simulink model "hrg_tdm_shared"  (R2025a)
settings: Solver=FixedStepDiscrete  StartTime=0.0  StopTime=c.duration  FixedStep=c.Ts  RelTol=1e-3
model workspace (MAT data in the model file):
  c.reuse = 1
  c.Ts = 6.25e-06
  c.w = 6283.18530718
  c.omega = 0.5
  c.duration = 1.2
  c.B = 0.276990961962
  c.driveEnd = 160
  c.senseStart = 192
  c.validStart = 272
  c.validEnd = 432
  c.frame = 480
  c.n = 160
  c.adcStep = 1.90734863281e-06
  c.adcMax = 0.999998092651
  c.adcMin = -1
  c.dacStep = 7.62939453125e-06
  c.dacMax = 0.999992370605
  c.dacMin = -1
  c.minEnergy = 0.0004
  c.minLinearity = 0.1
  c.agc = 12.5663706144
  c.gamma = 0.314159265359
  c.quad = 25.1327412287
  c.forceScale = 0.342719198573
  c.startCommand = [0; 0; 0; 0]
  c.pickoff = [0  0  0  0  0  0  0  0  0  0  0.1  0; 0  0  0  0  0  0  0  0  0  0  0  0.1]
  c.electrode = [0  0  0  0  0  0  6.28318530718e-05  0  0  0  0  0; 0  0  0  0  0  0  0  6.28318530718e-05  0  0  0  0]
  c.motion = [1  0  0  0  0  0  0  0  0  0  0  0; 0  1  0  0  0  0  0  0  0  0  0  0]
  c.Ad = [0.99922903725  -8.89767021045e-10  0.0392597386726  6.79661603948e-08  1.94082542713e-06  -5.91938484731e-08  0  0  0  0  0  0; 8.89767021045e-10  0.99922903725  -6.79661603948e-08  0.0392597386726  3.88142106306e-08  2.13106904302e-06  0  0  0  0  0  0; -0.0392597386726  -6.79661603967e-08  0.99922511127  3.46059382687e-06  9.39460935417e-05  -2.88897470742e-06  0  0  0  0  0  0; 6.79661603967e-08  -0.0392597386726  -3.46059382687e-06  0.99922511127  1.87875070496e-06  0.000104009857967  0  0  0  0  0  0; 0  0  0  0  0.731615628947  0  0  0  0  0  0  0; 0  0  0  0  0  0.770730381232  0  0  0  0  0  0; 0  0  0  0  11644.024379  0  0  0  0  0  0  0; 0  0  0  0  0  12266.5549964  0  0  0  0  0  0; 0  0  0  0  0  0  0  0  0.999937501953  0  0  0; 0  0  0  0  0  0  0  0  0  0.999937501953  0  0; 0  0  0  0  0  0  0  0  0.544042667727  0.0136010666932  0.455938127766  0; 0  0  0  0  0  0  0  0  -0.00760186665633  0.527062754839  0  0.493191201703]
  c.Bd = [2.07333228059e-07  -5.2482321733e-09; 4.14648229472e-09  1.8894232541e-07; 1.54445980203e-05  -3.92541399381e-07; 3.08873674204e-07  1.41320905111e-05; 0.268384371053  0; 0  0.229269618768; 4271.46993018  0; 0  3648.93931278; 0  0; 0  0; 0  0; 0  0]
  c.Af = [0.999229037252  -8.89767017797e-10  0.0392597384416  6.79661599867e-08  0  0  1.0729670464e-10  1.28007724625e-16  0  0  0  0; 8.89767017797e-10  0.999229037252  -6.79661599867e-08  0.0392597384416  0  0  -1.28007724618e-16  1.07296704251e-10  0  0  0  0; -0.0392597384416  -6.79661599886e-08  0.999225094196  3.46059378613e-06  0  0  5.10992633221e-09  9.4589441098e-15  0  0  0  0; 6.79661599886e-08  -0.0392597384416  -3.46059378613e-06  0.999225094196  0  0  -9.45894412526e-15  5.10992631239e-09  0  0  0  0; 0  0  0  0  0.731615628947  0  0  0  0  0  0  0; 0  0  0  0  0  0.770730381232  0  0  0  0  0  0; 0.107296704687  1.28007724925e-07  -5.10992633457  -9.45894414256e-06  0  0  0.65924020331  -1.83788136052e-14  0  0  0  0; -1.28007724925e-07  0.107296704687  9.45894414256e-06  -5.10992633457  0  0  1.83788135899e-14  0.65924020331  0  0  0  0; 0  0  0  0  0  0  0  0  0.731615628947  0  0  0; 0  0  0  0  0  0  0  0  0  0.731615628947  0  0; 0  0  0  0  0  0  0  0  0.457850378529  0.0114462594632  0.455938127766  0; 0  0  0  0  0  0  0  0  -0.00641037388191  0.444452589146  0  0.493191201703]
  c.As = [0.999229037251  -8.89767019419e-10  0.0392597385829  6.7966160211e-08  0  0  3.299223447e-11  4.96927081282e-17  0  0  0  0; 8.89767019419e-10  0.999229037251  -6.7966160211e-08  0.0392597385829  0  0  -4.9692697e-17  3.29922429769e-11  0  0  0  0; -0.0392597385829  -6.79661602128e-08  0.99922510602  3.46059381106e-06  0  0  9.97502201431e-10  2.90830921925e-15  0  0  0  0; 6.79661602128e-08  -0.0392597385829  -3.46059381106e-06  0.99922510602  0  0  -2.90830846447e-15  9.97502498523e-10  0  0  0  0; 0  0  0  0  0.731615628947  0  0  0  0  0  0  0; 0  0  0  0  0  0.770730381232  0  0  0  0  0  0; 0.0329922423735  4.96927093775e-08  -0.997502477449  -2.90830923686e-06  0  0  0.00193045194409  -2.36252148067e-15  0  0  0  0; -4.96927093775e-08  0.0329922423735  2.90830923686e-06  -0.997502477449  0  0  2.36252088829e-15  0.00193045194409  0  0  0  0; 0.000563655894429  5.77530332379e-10  -0.0329913452873  -4.96917902079e-08  0  0  0.00627072528027  -3.48479736566e-17  0.999937501953  0  0  0; -5.77530332379e-10  0.000563655894429  4.96917902079e-08  -0.0329913452873  0  0  3.4847965996e-17  0.00627072528027  0  0.999937501953  0  0; 0.000110797632844  2.77002999452e-06  -0.00905716494292  -0.000226438897931  0  0  0.00300835962776  7.52089906939e-05  0.544042667727  0.0136010666932  0.455938127766  0; -1.51991580376e-06  0.000105374968441  0.000124839418396  -0.00865488875584  0  0  -4.18601716323e-05  0.00290230523317  -0.00760186665633  0.527062754839  0  0.493191201703]
  c.x0 = [0.276318298201; 0.116825502693; 0; 0; 0; 0; 0; 0; 0; 0; 0; 0]
  c.detect = [-9.99415152174  0.240237763684  -0.546724271016  0.0144774125637; -0.144146416179  -9.60951054736  -0.00788544621657  -0.579096502547; 0.546724271016  -0.0144774125637  -9.99415152174  0.240237763684; 0.00788544621657  0.579096502547  -0.144146416179  -9.60951054736]
  c.drive = [0.996850279412  0.0276902855392  0.14520184302  0.00403338452835; -0.018451056911  0.922552845551  -0.00315402594922  0.157701297461; -0.14520184302  -0.00403338452835  0.996850279412  0.0276902855392; 0.00315402594922  -0.157701297461  -0.018451056911  0.922552845551]
settings Model: Creator=Administrator  LastModifiedBy=Administrator

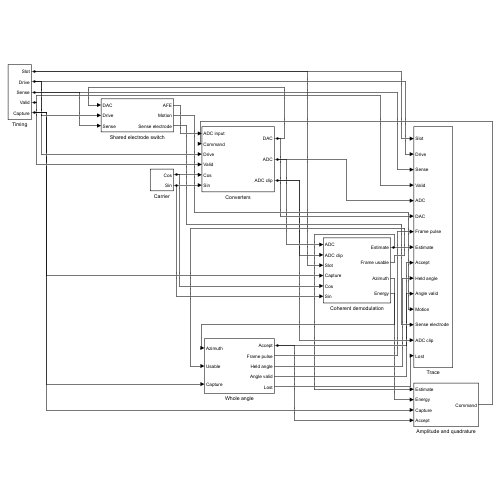
[thumbnail: Simulink's stored preview of the top-level diagram]
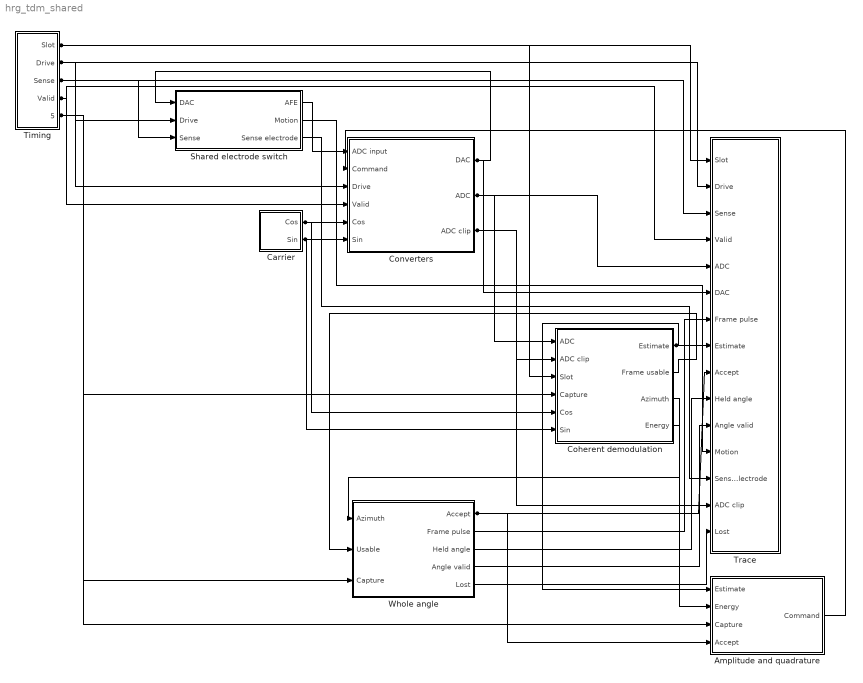
== system hrg_tdm_shared ==
  Amplitude and quadrature : Subsystem
  Carrier : Subsystem
  Coherent demodulation : Subsystem
  Converters : Subsystem
  Shared electrode switch : Subsystem
  Timing : Subsystem
  Trace : Subsystem
  Whole angle : Subsystem
  wires:
  Timing/1(Slot) -> Trace/1(Slot), Coherent demodulation/3(Slot)
  Timing/2(Drive) -> Trace/2(Drive), Converters/3(Drive), Shared electrode switch/2(Drive)
  Timing/3(Sense) -> Trace/3(Sense), Shared electrode switch/3(Sense)
  Coherent demodulation/2(Frame usable) -> Whole angle/2(Usable)
  Shared electrode switch/2(Motion) -> Trace/12(Motion)
  Shared electrode switch/1(AFE) -> Converters/1(ADC input)
  Carrier/2(Sin) -> Coherent demodulation/6(Sin), Converters/6(Sin)
  Timing/4(Valid) -> Converters/4(Valid), Trace/4(Valid)
  Whole angle/1(Accept) -> Trace/9(Accept), Amplitude and quadrature/4(Accept)
  Timing/5(Capture) -> Coherent demodulation/4(Capture), Amplitude and quadrature/3(Capture), Whole angle/3(Capture)
  Shared electrode switch/3(Sense electrode) -> Trace/13(Sense electrode)
  Carrier/1(Cos) -> Coherent demodulation/5(Cos), Converters/5(Cos)
  Converters/1(DAC) -> Shared electrode switch/1(DAC), Trace/6(DAC)
  Converters/2(ADC) -> Trace/5(ADC), Coherent demodulation/1(ADC)
  Converters/3(ADC clip) -> Trace/14(ADC clip), Coherent demodulation/2(ADC clip)
  Whole angle/2(Frame pulse) -> Trace/7(Frame pulse)
  Whole angle/3(Held angle) -> Trace/10(Held angle)
  Coherent demodulation/1(Estimate) -> Amplitude and quadrature/1(Estimate), Trace/8(Estimate)
  Whole angle/4(Angle valid) -> Trace/11(Angle valid)
  Whole angle/5(Lost) -> Trace/15(Lost)
  Coherent demodulation/3(Azimuth) -> Whole angle/1(Azimuth)
  Coherent demodulation/4(Energy) -> Amplitude and quadrature/2(Energy)
  Amplitude and quadrature/1(Command) -> Converters/2(Command)

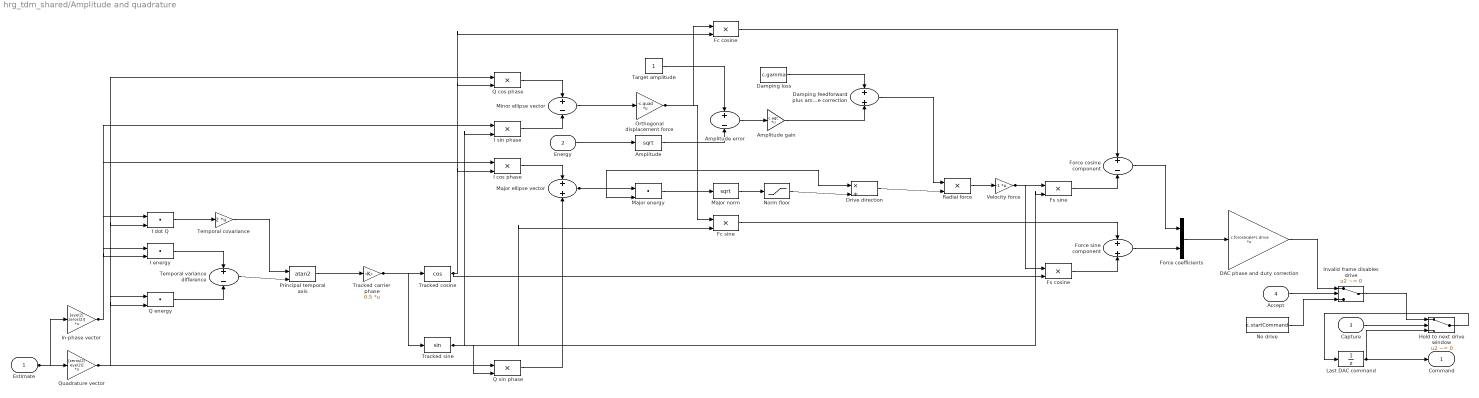
== system hrg_tdm_shared/Amplitude and quadrature ==
  Estimate : Inport
  Energy : Inport  Port=2
  Capture : Inport  Port=3
  Accept : Inport  Port=4
  Amplitude : Sqrt
  Amplitude error : Sum  Inputs=+-
  Amplitude gain : Gain  Gain=c.agc  Multiplication=Matrix(K*u)
  DAC phase and duty correction : Gain  Gain=c.forceScale*c.drive  Multiplication=Matrix(K*u)
  Damping feedforward plus amplitude correction : Sum
  Damping loss : Constant  Value=c.gamma
  Drive direction : Product  Inputs=*/
  Fc cosine : Product
  Fc sine : Product
  Force coefficients : Mux  Inputs=2
  Force cosine component : Sum  Inputs=+-
  Force sine component : Sum
  Fs cosine : Product
  Fs sine : Product
  Hold to next drive window : Switch  Criteria=u2 ~= 0  SaturateOnIntegerOverflow=off  InputSameDT=off
  I cos phase : Product
  I dot Q : DotProduct  OutDataTypeStr=Inherit: Inherit via internal rule
  I energy : DotProduct  OutDataTypeStr=Inherit: Inherit via internal rule
  I sin phase : Product
  In-phase vector : Gain  Gain=[eye(2) zeros(2)]  Multiplication=Matrix(K*u)
  Invalid frame disables drive : Switch  Criteria=u2 ~= 0  SaturateOnIntegerOverflow=off  InputSameDT=off
  Last DAC command : UnitDelay  InitialCondition=c.startCommand  SampleTime=c.Ts  HasFrameUpgradeWarning=on
  Major ellipse vector : Sum
  Major energy : DotProduct  OutDataTypeStr=Inherit: Inherit via internal rule
  Major norm : Sqrt
  Minor ellipse vector : Sum  Inputs=+-
  No drive : Constant  Value=c.startCommand
  Norm floor : Saturate  UpperLimit=inf  LowerLimit=1e-9
  Orthogonal displacement force : Gain  Gain=-c.quad  Multiplication=Matrix(K*u)
  Principal temporal axis : Trigonometry  Operator=atan2
  Q cos phase : Product
  Q energy : DotProduct  OutDataTypeStr=Inherit: Inherit via internal rule
  Q sin phase : Product
  Quadrature vector : Gain  Gain=[zeros(2) eye(2)]  Multiplication=Matrix(K*u)
  Radial force : Product
  Target amplitude : Constant
  Temporal covariance : Gain  Gain=2  Multiplication=Matrix(K*u)
  Temporal variance difference : Sum  Inputs=+-
  Tracked carrier phase : Gain  Gain=0.5  Multiplication=Matrix(K*u)
  Tracked cosine : Trigonometry  Operator=cos
  Tracked sine : Trigonometry
  Velocity force : Gain  Gain=-1  Multiplication=Matrix(K*u)
  Command : Outport
  wires:
  Estimate/1 -> In-phase vector/1, Quadrature vector/1
  Temporal covariance/1 -> Principal temporal axis/1
  I dot Q/1 -> Temporal covariance/1
  In-phase vector/1 -> I sin phase/1, I energy/1, I energy/2, I dot Q/1, I cos phase/1
  Amplitude gain/1 -> Damping feedforward plus amplitude correction/2
  Tracked carrier phase/1 -> Tracked cosine/1, Tracked sine/1
  Temporal variance difference/1 -> Principal temporal axis/2
  Minor ellipse vector/1 -> Orthogonal displacement force/1
  Quadrature vector/1 -> Q sin phase/1, Q cos phase/1, Q energy/1, Q energy/2, I dot Q/2
  Force coefficients/1 -> DAC phase and duty correction/1
  I energy/1 -> Temporal variance difference/1
  Q energy/1 -> Temporal variance difference/2
  Principal temporal axis/1 -> Tracked carrier phase/1
  Force sine component/1 -> Force coefficients/2
  Tracked cosine/1 -> Fc cosine/2, Fs cosine/2, Q cos phase/2, I cos phase/2
  Energy/1 -> Amplitude/1
  Tracked sine/1 -> Fc sine/2, Fs sine/2, I sin phase/2, Q sin phase/2
  No drive/1 -> Invalid frame disables drive/3
  Fs cosine/1 -> Force sine component/2
  Q cos phase/1 -> Minor ellipse vector/1
  Amplitude error/1 -> Amplitude gain/1
  I sin phase/1 -> Minor ellipse vector/2
  I cos phase/1 -> Major ellipse vector/1
  Q sin phase/1 -> Major ellipse vector/2
  DAC phase and duty correction/1 -> Invalid frame disables drive/1
  Major ellipse vector/1 -> Drive direction/1, Major energy/1, Major energy/2
  Capture/1 -> Hold to next drive window/2
  Fc cosine/1 -> Force cosine component/1
  Target amplitude/1 -> Amplitude error/1
  Orthogonal displacement force/1 -> Fc sine/1, Fc cosine/1
  Amplitude/1 -> Amplitude error/2
  Major energy/1 -> Major norm/1
  Major norm/1 -> Norm floor/1
  Fc sine/1 -> Force sine component/1
  Force cosine component/1 -> Force coefficients/1
  Damping loss/1 -> Damping feedforward plus amplitude correction/1
  Norm floor/1 -> Drive direction/2
  Damping feedforward plus amplitude correction/1 -> Radial force/1
  Drive direction/1 -> Radial force/2
  Radial force/1 -> Velocity force/1
  Velocity force/1 -> Fs sine/1, Fs cosine/1
  Fs sine/1 -> Force cosine component/2
  Accept/1 -> Invalid frame disables drive/2
  Invalid frame disables drive/1 -> Hold to next drive window/1
  Last DAC command/1 -> Hold to next drive window/3, Command/1
  Hold to next drive window/1 -> Last DAC command/1

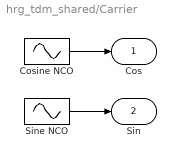
== system hrg_tdm_shared/Carrier ==
  Cosine NCO : Sin  Frequency=c.w  Phase=pi/2  SampleTime=c.Ts
  Sine NCO : Sin  Frequency=c.w  SampleTime=c.Ts
  Cos : Outport
  Sin : Outport  Port=2
  wires:
  Cosine NCO/1 -> Cos/1
  Sine NCO/1 -> Sin/1

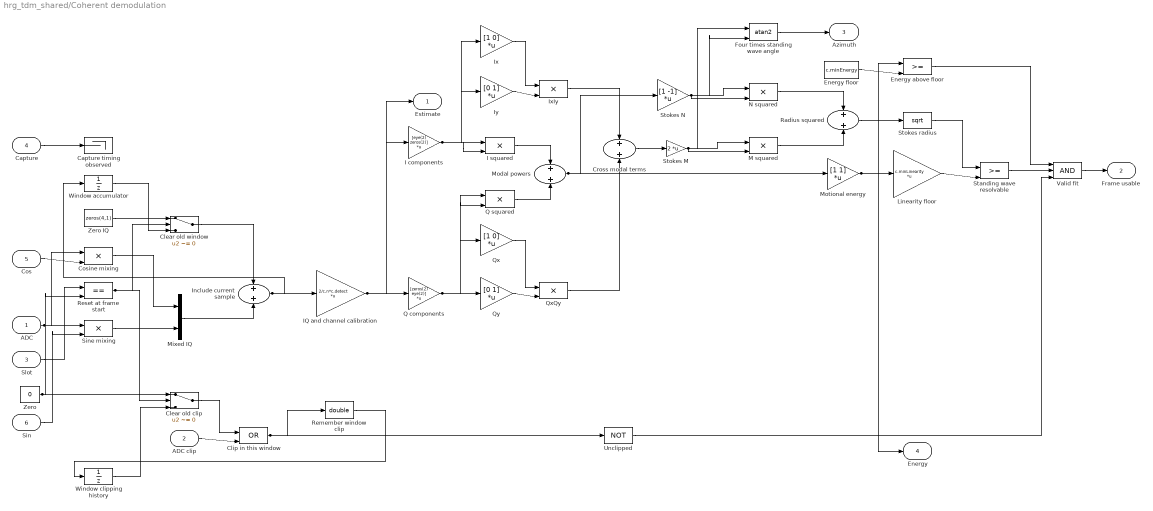
== system hrg_tdm_shared/Coherent demodulation ==
  ADC : Inport
  ADC clip : Inport  Port=2
  Slot : Inport  Port=3
  Capture : Inport  Port=4
  Cos : Inport  Port=5
  Sin : Inport  Port=6
  Capture timing observed : Terminator
  Clear old clip : Switch  Criteria=u2 ~= 0  SaturateOnIntegerOverflow=off  InputSameDT=off
  Clear old window : Switch  Criteria=u2 ~= 0  SaturateOnIntegerOverflow=off  InputSameDT=off
  Clip in this window : Logic  Operator=OR  AllPortsSameDT=off  OutDataTypeStr=boolean
  Cosine mixing : Product
  Cross modal terms : Sum
  Energy above floor : RelationalOperator  OutDataTypeStr=boolean  RndMeth=Simplest  InputSameDT=off
  Energy floor : Constant  Value=c.minEnergy
  Four times standing wave angle : Trigonometry  Operator=atan2
  I components : Gain  Gain=[eye(2) zeros(2)]  Multiplication=Matrix(K*u)
  I squared : Product
  IQ and channel calibration : Gain  Gain=2/c.n*c.detect  Multiplication=Matrix(K*u)
  Include current sample : Sum
  Ix : Gain  Gain=[1 0]  Multiplication=Matrix(K*u)
  IxIy : Product
  Iy : Gain  Gain=[0 1]  Multiplication=Matrix(K*u)
  Linearity floor : Gain  Gain=c.minLinearity  Multiplication=Matrix(K*u)
  M squared : Product
  Mixed IQ : Mux  Inputs=2
  Modal powers : Sum
  Motional energy : Gain  Gain=[1 1]  Multiplication=Matrix(K*u)
  N squared : Product
  Q components : Gain  Gain=[zeros(2) eye(2)]  Multiplication=Matrix(K*u)
  Q squared : Product
  Qx : Gain  Gain=[1 0]  Multiplication=Matrix(K*u)
  QxQy : Product
  Qy : Gain  Gain=[0 1]  Multiplication=Matrix(K*u)
  Radius squared : Sum
  Remember window clip : DataTypeConversion  OutDataTypeStr=double  SaturateOnIntegerOverflow=off  RndMeth=Floor
  Reset at frame start : RelationalOperator  Operator===  OutDataTypeStr=boolean  RndMeth=Simplest  InputSameDT=off
  Sine mixing : Product
  Standing wave resolvable : RelationalOperator  OutDataTypeStr=boolean  RndMeth=Simplest  InputSameDT=off
  Stokes M : Gain  Gain=2  Multiplication=Matrix(K*u)
  Stokes N : Gain  Gain=[1 -1]  Multiplication=Matrix(K*u)
  Stokes radius : Sqrt
  Unclipped : Logic  Operator=NOT  Inputs=1  AllPortsSameDT=off  OutDataTypeStr=boolean
  Valid fit : Logic  Inputs=3  AllPortsSameDT=off  OutDataTypeStr=boolean
  Window accumulator : UnitDelay  InitialCondition=zeros(4,1)  SampleTime=c.Ts  HasFrameUpgradeWarning=on
  Window clipping history : UnitDelay  SampleTime=c.Ts  HasFrameUpgradeWarning=on
  Zero : Constant  Value=0
  Zero IQ : Constant  Value=zeros(4,1)
  Estimate : Outport
  Frame usable : Outport  Port=2
  Azimuth : Outport  Port=3
  Energy : Outport  Port=4
  wires:
  Slot/1 -> Reset at frame start/1
  I components/1 -> I squared/2, Ix/1, Iy/1, I squared/1
  Clear old clip/1 -> Clip in this window/1
  Capture/1 -> Capture timing observed/1
  I squared/1 -> Modal powers/1
  Cos/1 -> Cosine mixing/2
  Zero/1 -> Clear old clip/1, Reset at frame start/2
  Stokes radius/1 -> Standing wave resolvable/1
  ADC/1 -> Cosine mixing/1, Sine mixing/1
  ADC clip/1 -> Clip in this window/2
  Sin/1 -> Sine mixing/2
  Window accumulator/1 -> Clear old window/3
  Cross modal terms/1 -> Stokes M/1
  Zero IQ/1 -> Clear old window/1
  Cosine mixing/1 -> Mixed IQ/1
  Reset at frame start/1 -> Clear old clip/2, Clear old window/2
  Standing wave resolvable/1 -> Valid fit/2
  Sine mixing/1 -> Mixed IQ/2
  Window clipping history/1 -> Clear old clip/3
  Clear old window/1 -> Include current sample/1
  Mixed IQ/1 -> Include current sample/2
  Motional energy/1 -> Energy above floor/1, Linearity floor/1, Energy/1
  Include current sample/1 -> Window accumulator/1, IQ and channel calibration/1
  Clip in this window/1 -> Unclipped/1, Remember window clip/1
  IQ and channel calibration/1 -> I components/1, Q components/1, Estimate/1
  Remember window clip/1 -> Window clipping history/1
  Q components/1 -> Q squared/1, Qy/1, Qx/1, Q squared/2
  Unclipped/1 -> Valid fit/3
  Ix/1 -> IxIy/1
  Iy/1 -> IxIy/2
  Q squared/1 -> Modal powers/2
  Qx/1 -> QxQy/1
  Linearity floor/1 -> Standing wave resolvable/2
  M squared/1 -> Radius squared/2
  Qy/1 -> QxQy/2
  IxIy/1 -> Cross modal terms/1
  Modal powers/1 -> Motional energy/1, Stokes N/1
  QxQy/1 -> Cross modal terms/2
  Stokes N/1 -> N squared/1, Four times standing wave angle/2, N squared/2
  Stokes M/1 -> Four times standing wave angle/1, M squared/1, M squared/2
  Four times standing wave angle/1 -> Azimuth/1
  N squared/1 -> Radius squared/1
  Energy floor/1 -> Energy above floor/2
  Radius squared/1 -> Stokes radius/1
  Energy above floor/1 -> Valid fit/1
  Valid fit/1 -> Frame usable/1

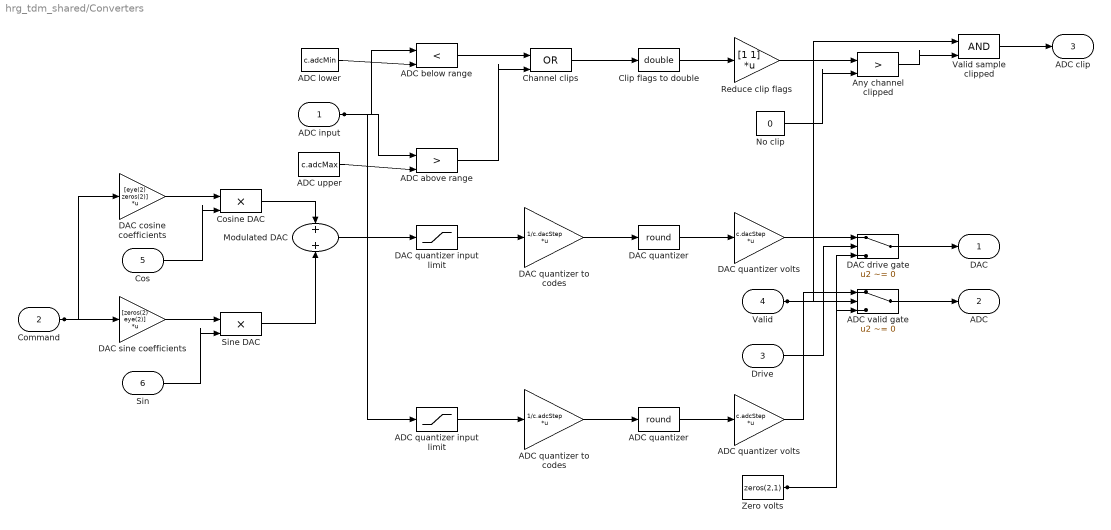
== system hrg_tdm_shared/Converters ==
  ADC input : Inport
  Command : Inport  Port=2
  Drive : Inport  Port=3
  Valid : Inport  Port=4
  Cos : Inport  Port=5
  Sin : Inport  Port=6
  ADC above range : RelationalOperator  Operator=>  OutDataTypeStr=boolean  RndMeth=Simplest  InputSameDT=off
  ADC below range : RelationalOperator  Operator=<  OutDataTypeStr=boolean  RndMeth=Simplest  InputSameDT=off
  ADC lower : Constant  Value=c.adcMin
  ADC quantizer : Rounding  Operator=round
  ADC quantizer input limit : Saturate  UpperLimit=c.adcMax  LowerLimit=c.adcMin
  ADC quantizer to codes : Gain  Gain=1/c.adcStep  Multiplication=Matrix(K*u)
  ADC quantizer volts : Gain  Gain=c.adcStep  Multiplication=Matrix(K*u)
  ADC upper : Constant  Value=c.adcMax
  ADC valid gate : Switch  Criteria=u2 ~= 0  SaturateOnIntegerOverflow=off  InputSameDT=off
  Any channel clipped : RelationalOperator  Operator=>  OutDataTypeStr=boolean  RndMeth=Simplest  InputSameDT=off
  Channel clips : Logic  Operator=OR  AllPortsSameDT=off  OutDataTypeStr=boolean
  Clip flags to double : DataTypeConversion  OutDataTypeStr=double  SaturateOnIntegerOverflow=off  RndMeth=Floor
  Cosine DAC : Product
  DAC cosine coefficients : Gain  Gain=[eye(2) zeros(2)]  Multiplication=Matrix(K*u)
  DAC drive gate : Switch  Criteria=u2 ~= 0  SaturateOnIntegerOverflow=off  InputSameDT=off
  DAC quantizer : Rounding  Operator=round
  DAC quantizer input limit : Saturate  UpperLimit=c.dacMax  LowerLimit=c.dacMin
  DAC quantizer to codes : Gain  Gain=1/c.dacStep  Multiplication=Matrix(K*u)
  DAC quantizer volts : Gain  Gain=c.dacStep  Multiplication=Matrix(K*u)
  DAC sine coefficients : Gain  Gain=[zeros(2) eye(2)]  Multiplication=Matrix(K*u)
  Modulated DAC : Sum
  No clip : Constant  Value=0
  Reduce clip flags : Gain  Gain=[1 1]  Multiplication=Matrix(K*u)
  Sine DAC : Product
  Valid sample clipped : Logic  AllPortsSameDT=off  OutDataTypeStr=boolean
  Zero volts : Constant  Value=zeros(2,1)
  DAC : Outport
  ADC : Outport  Port=2
  ADC clip : Outport  Port=3
  wires:
  Sine DAC/1 -> Modulated DAC/2
  Command/1 -> DAC cosine coefficients/1, DAC sine coefficients/1
  Cos/1 -> Cosine DAC/2
  DAC cosine coefficients/1 -> Cosine DAC/1
  Sin/1 -> Sine DAC/2
  DAC sine coefficients/1 -> Sine DAC/1
  Cosine DAC/1 -> Modulated DAC/1
  ADC lower/1 -> ADC below range/2
  ADC input/1 -> ADC quantizer input limit/1, ADC below range/1, ADC above range/1
  Valid sample clipped/1 -> ADC clip/1
  ADC upper/1 -> ADC above range/2
  Any channel clipped/1 -> Valid sample clipped/2
  Modulated DAC/1 -> DAC quantizer input limit/1
  ADC quantizer to codes/1 -> ADC quantizer/1
  ADC below range/1 -> Channel clips/1
  Valid/1 -> Valid sample clipped/1, ADC valid gate/2
  ADC above range/1 -> Channel clips/2
  Clip flags to double/1 -> Reduce clip flags/1
  DAC quantizer input limit/1 -> DAC quantizer to codes/1
  ADC quantizer input limit/1 -> ADC quantizer to codes/1
  Channel clips/1 -> Clip flags to double/1
  DAC quantizer volts/1 -> DAC drive gate/1
  Reduce clip flags/1 -> Any channel clipped/1
  DAC quantizer to codes/1 -> DAC quantizer/1
  DAC quantizer/1 -> DAC quantizer volts/1
  ADC quantizer/1 -> ADC quantizer volts/1
  No clip/1 -> Any channel clipped/2
  Drive/1 -> DAC drive gate/2
  ADC quantizer volts/1 -> ADC valid gate/1
  Zero volts/1 -> DAC drive gate/3, ADC valid gate/3
  DAC drive gate/1 -> DAC/1
  ADC valid gate/1 -> ADC/1

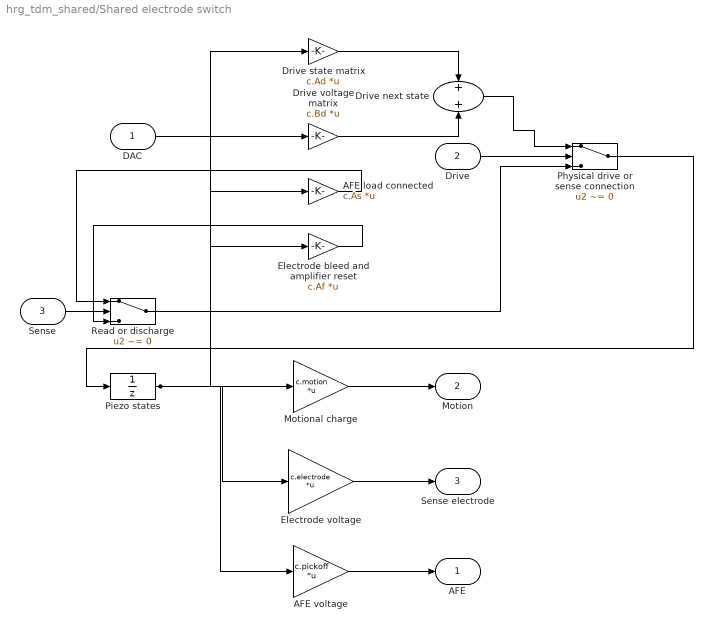
== system hrg_tdm_shared/Shared electrode switch ==
  DAC : Inport
  Drive : Inport  Port=2
  Sense : Inport  Port=3
  AFE load connected : Gain  Gain=c.As  Multiplication=Matrix(K*u)
  AFE voltage : Gain  Gain=c.pickoff  Multiplication=Matrix(K*u)
  Drive next state : Sum
  Drive state matrix : Gain  Gain=c.Ad  Multiplication=Matrix(K*u)
  Drive voltage matrix : Gain  Gain=c.Bd  Multiplication=Matrix(K*u)
  Electrode bleed and amplifier reset : Gain  Gain=c.Af  Multiplication=Matrix(K*u)
  Electrode voltage : Gain  Gain=c.electrode  Multiplication=Matrix(K*u)
  Motional charge : Gain  Gain=c.motion  Multiplication=Matrix(K*u)
  Physical drive or sense connection : Switch  Criteria=u2 ~= 0  SaturateOnIntegerOverflow=off  InputSameDT=off
  Piezo states : UnitDelay  InitialCondition=c.x0  SampleTime=c.Ts  HasFrameUpgradeWarning=on
  Read or discharge : Switch  Criteria=u2 ~= 0  SaturateOnIntegerOverflow=off  InputSameDT=off
  AFE : Outport
  Motion : Outport  Port=2
  Sense electrode : Outport  Port=3
  wires:
  Electrode bleed and amplifier reset/1 -> Read or discharge/3
  Drive state matrix/1 -> Drive next state/1
  DAC/1 -> Drive voltage matrix/1
  Sense/1 -> Read or discharge/2
  Read or discharge/1 -> Physical drive or sense connection/3
  Piezo states/1 -> Drive state matrix/1, Electrode bleed and amplifier reset/1, AFE load connected/1, AFE voltage/1, Electrode voltage/1, Motional charge/1
  Drive voltage matrix/1 -> Drive next state/2
  AFE load connected/1 -> Read or discharge/1
  Motional charge/1 -> Motion/1
  Electrode voltage/1 -> Sense electrode/1
  AFE voltage/1 -> AFE/1
  Drive next state/1 -> Physical drive or sense connection/1
  Drive/1 -> Physical drive or sense connection/2
  Physical drive or sense connection/1 -> Piezo states/1

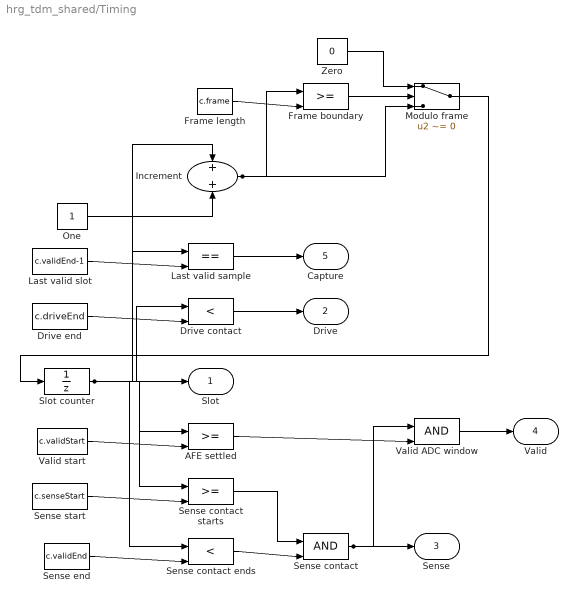
== system hrg_tdm_shared/Timing ==
  AFE settled : RelationalOperator  OutDataTypeStr=boolean  RndMeth=Simplest  InputSameDT=off
  Drive contact : RelationalOperator  Operator=<  OutDataTypeStr=boolean  RndMeth=Simplest  InputSameDT=off
  Drive end : Constant  Value=c.driveEnd
  Frame boundary : RelationalOperator  OutDataTypeStr=boolean  RndMeth=Simplest  InputSameDT=off
  Frame length : Constant  Value=c.frame
  Increment : Sum
  Last valid sample : RelationalOperator  Operator===  OutDataTypeStr=boolean  RndMeth=Simplest  InputSameDT=off
  Last valid slot : Constant  Value=c.validEnd-1
  Modulo frame : Switch  Criteria=u2 ~= 0  SaturateOnIntegerOverflow=off  InputSameDT=off
  One : Constant
  Sense contact : Logic  AllPortsSameDT=off  OutDataTypeStr=boolean
  Sense contact ends : RelationalOperator  Operator=<  OutDataTypeStr=boolean  RndMeth=Simplest  InputSameDT=off
  Sense contact starts : RelationalOperator  OutDataTypeStr=boolean  RndMeth=Simplest  InputSameDT=off
  Sense end : Constant  Value=c.validEnd
  Sense start : Constant  Value=c.senseStart
  Slot counter : UnitDelay  SampleTime=c.Ts  HasFrameUpgradeWarning=on
  Valid ADC window : Logic  AllPortsSameDT=off  OutDataTypeStr=boolean
  Valid start : Constant  Value=c.validStart
  Zero : Constant  Value=0
  Slot : Outport
  Drive : Outport  Port=2
  Sense : Outport  Port=3
  Valid : Outport  Port=4
  Capture : Outport  Port=5
  wires:
  One/1 -> Increment/2
  Last valid slot/1 -> Last valid sample/2
  Drive end/1 -> Drive contact/2
  Frame length/1 -> Frame boundary/2
  Slot counter/1 -> Increment/1, Drive contact/1, AFE settled/1, Sense contact ends/1, Sense contact starts/1, Last valid sample/1, Slot/1
  Valid start/1 -> AFE settled/2
  Last valid sample/1 -> Capture/1
  Sense end/1 -> Sense contact ends/2
  Sense start/1 -> Sense contact starts/2
  Increment/1 -> Modulo frame/3, Frame boundary/1
  Drive contact/1 -> Drive/1
  AFE settled/1 -> Valid ADC window/2
  Sense contact starts/1 -> Sense contact/1
  Sense contact ends/1 -> Sense contact/2
  Zero/1 -> Modulo frame/1
  Frame boundary/1 -> Modulo frame/2
  Sense contact/1 -> Valid ADC window/1, Sense/1
  Valid ADC window/1 -> Valid/1
  Modulo frame/1 -> Slot counter/1

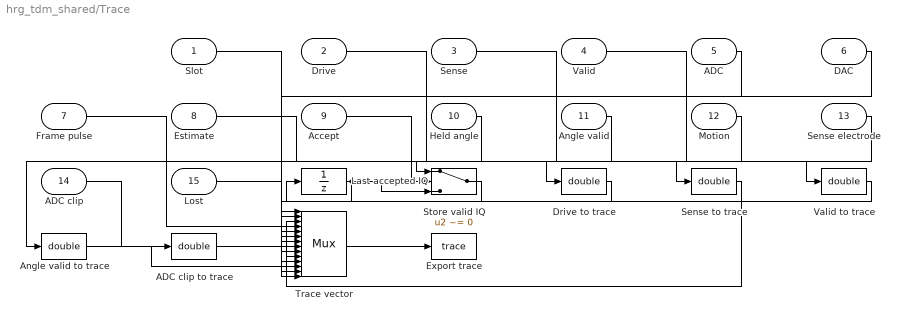
== system hrg_tdm_shared/Trace ==
  Slot : Inport
  Drive : Inport  Port=2
  Sense : Inport  Port=3
  Valid : Inport  Port=4
  ADC : Inport  Port=5
  DAC : Inport  Port=6
  Frame pulse : Inport  Port=7
  Estimate : Inport  Port=8
  Accept : Inport  Port=9
  Held angle : Inport  Port=10
  Angle valid : Inport  Port=11
  Motion : Inport  Port=12
  Sense electrode : Inport  Port=13
  ADC clip : Inport  Port=14
  Lost : Inport  Port=15
  ADC clip to trace : DataTypeConversion  OutDataTypeStr=double  SaturateOnIntegerOverflow=off  RndMeth=Floor
  Angle valid to trace : DataTypeConversion  OutDataTypeStr=double  SaturateOnIntegerOverflow=off  RndMeth=Floor
  Drive to trace : DataTypeConversion  OutDataTypeStr=double  SaturateOnIntegerOverflow=off  RndMeth=Floor
  Export trace : ToWorkspace  VariableName=trace  SampleTime=-1
  Last accepted IQ : UnitDelay  InitialCondition=zeros(4,1)  SampleTime=c.Ts  HasFrameUpgradeWarning=on
  Sense to trace : DataTypeConversion  OutDataTypeStr=double  SaturateOnIntegerOverflow=off  RndMeth=Floor
  Store valid IQ : Switch  Criteria=u2 ~= 0  SaturateOnIntegerOverflow=off  InputSameDT=off
  Trace vector : Mux  Inputs=14
  Valid to trace : DataTypeConversion  OutDataTypeStr=double  SaturateOnIntegerOverflow=off  RndMeth=Floor
  wires:
  Estimate/1 -> Store valid IQ/1
  Accept/1 -> Store valid IQ/2
  Last accepted IQ/1 -> Store valid IQ/3, Trace vector/8
  Store valid IQ/1 -> Last accepted IQ/1
  Drive/1 -> Drive to trace/1
  Sense/1 -> Sense to trace/1
  Valid/1 -> Valid to trace/1
  Angle valid/1 -> Angle valid to trace/1
  ADC clip/1 -> ADC clip to trace/1
  Slot/1 -> Trace vector/1
  Drive to trace/1 -> Trace vector/2
  Sense to trace/1 -> Trace vector/3
  Valid to trace/1 -> Trace vector/4
  ADC/1 -> Trace vector/5
  DAC/1 -> Trace vector/6
  Frame pulse/1 -> Trace vector/7
  Held angle/1 -> Trace vector/9
  Angle valid to trace/1 -> Trace vector/10
  Motion/1 -> Trace vector/11
  Sense electrode/1 -> Trace vector/12
  ADC clip to trace/1 -> Trace vector/13
  Lost/1 -> Trace vector/14
  Trace vector/1 -> Export trace/1

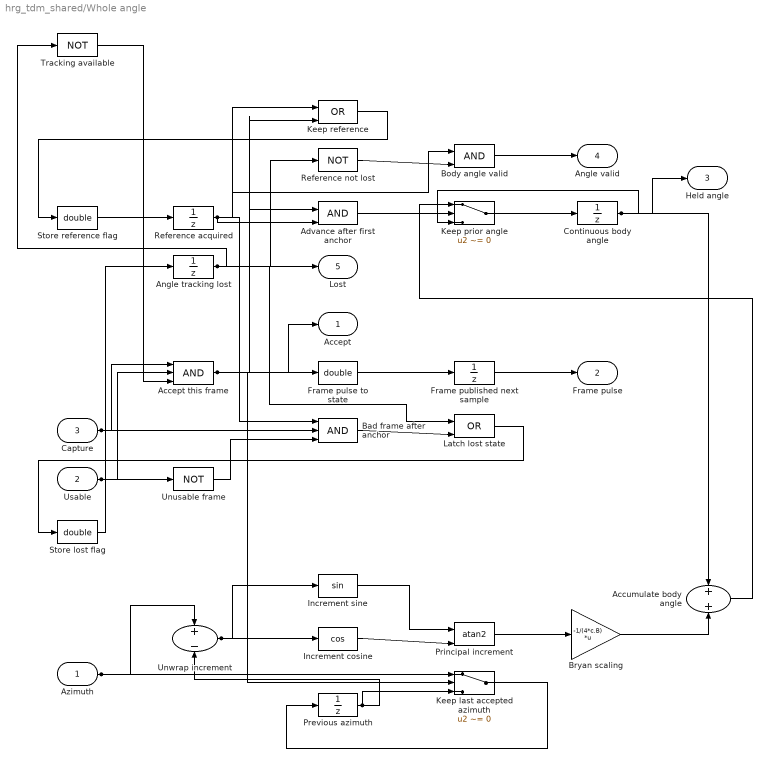
== system hrg_tdm_shared/Whole angle ==
  Azimuth : Inport
  Usable : Inport  Port=2
  Capture : Inport  Port=3
  Accept this frame : Logic  Inputs=3  AllPortsSameDT=off  OutDataTypeStr=boolean
  Accumulate body angle : Sum
  Advance after first anchor : Logic  AllPortsSameDT=off  OutDataTypeStr=boolean
  Angle tracking lost : UnitDelay  SampleTime=c.Ts  HasFrameUpgradeWarning=on
  Bad frame after anchor : Logic  Inputs=3  AllPortsSameDT=off  OutDataTypeStr=boolean
  Body angle valid : Logic  AllPortsSameDT=off  OutDataTypeStr=boolean
  Bryan scaling : Gain  Gain=-1/(4*c.B)  Multiplication=Matrix(K*u)
  Continuous body angle : UnitDelay  SampleTime=c.Ts  HasFrameUpgradeWarning=on
  Frame published next sample : UnitDelay  SampleTime=c.Ts  HasFrameUpgradeWarning=on
  Frame pulse to state : DataTypeConversion  OutDataTypeStr=double  SaturateOnIntegerOverflow=off  RndMeth=Floor
  Increment cosine : Trigonometry  Operator=cos
  Increment sine : Trigonometry
  Keep last accepted azimuth : Switch  Criteria=u2 ~= 0  SaturateOnIntegerOverflow=off  InputSameDT=off
  Keep prior angle : Switch  Criteria=u2 ~= 0  SaturateOnIntegerOverflow=off  InputSameDT=off
  Keep reference : Logic  Operator=OR  AllPortsSameDT=off  OutDataTypeStr=boolean
  Latch lost state : Logic  Operator=OR  AllPortsSameDT=off  OutDataTypeStr=boolean
  Previous azimuth : UnitDelay  SampleTime=c.Ts  HasFrameUpgradeWarning=on
  Principal increment : Trigonometry  Operator=atan2
  Reference acquired : UnitDelay  SampleTime=c.Ts  HasFrameUpgradeWarning=on
  Reference not lost : Logic  Operator=NOT  Inputs=1  AllPortsSameDT=off  OutDataTypeStr=boolean
  Store lost flag : DataTypeConversion  OutDataTypeStr=double  SaturateOnIntegerOverflow=off  RndMeth=Floor
  Store reference flag : DataTypeConversion  OutDataTypeStr=double  SaturateOnIntegerOverflow=off  RndMeth=Floor
  Tracking available : Logic  Operator=NOT  Inputs=1  AllPortsSameDT=off  OutDataTypeStr=boolean
  Unusable frame : Logic  Operator=NOT  Inputs=1  AllPortsSameDT=off  OutDataTypeStr=boolean
  Unwrap increment : Sum  Inputs=+-
  Accept : Outport
  Frame pulse : Outport  Port=2
  Held angle : Outport  Port=3
  Angle valid : Outport  Port=4
  Lost : Outport  Port=5
  wires:
  Store reference flag/1 -> Reference acquired/1
  Tracking available/1 -> Accept this frame/3
  Capture/1 -> Bad frame after anchor/2, Accept this frame/1
  Reference acquired/1 -> Keep reference/1, Bad frame after anchor/1, Advance after first anchor/2, Body angle valid/1
  Usable/1 -> Accept this frame/2, Unusable frame/1
  Reference not lost/1 -> Body angle valid/2
  Azimuth/1 -> Keep last accepted azimuth/1, Unwrap increment/1
  Store lost flag/1 -> Angle tracking lost/1
  Angle tracking lost/1 -> Latch lost state/1, Tracking available/1, Reference not lost/1, Lost/1
  Accept this frame/1 -> Keep last accepted azimuth/2, Frame pulse to state/1, Keep reference/2, Advance after first anchor/1, Accept/1
  Unusable frame/1 -> Bad frame after anchor/3
  Unwrap increment/1 -> Increment sine/1, Increment cosine/1
  Keep last accepted azimuth/1 -> Previous azimuth/1
  Keep reference/1 -> Store reference flag/1
  Advance after first anchor/1 -> Keep prior angle/2
  Frame pulse to state/1 -> Frame published next sample/1
  Bad frame after anchor/1 -> Latch lost state/2
  Increment sine/1 -> Principal increment/1
  Increment cosine/1 -> Principal increment/2
  Previous azimuth/1 -> Unwrap increment/2, Keep last accepted azimuth/3
  Body angle valid/1 -> Angle valid/1
  Continuous body angle/1 -> Accumulate body angle/1, Held angle/1, Keep prior angle/3
  Keep prior angle/1 -> Continuous body angle/1
  Frame published next sample/1 -> Frame pulse/1
  Latch lost state/1 -> Store lost flag/1
  Principal increment/1 -> Bryan scaling/1
  Bryan scaling/1 -> Accumulate body angle/2
  Accumulate body angle/1 -> Keep prior angle/1
